simulink model "r2_b16a4x64f"  (R2012b)
settings: Solver=VariableStepDiscrete  SolverMode=SingleTasking  StartTime=0.0  StopTime=1  RelTol=1e-3
undefined symbols (not defined in the file): fft_stages, n_bits_ants, n_bits_xengs
libraries: xbsIndex_r4 x26846, casper_library_misc x230, xbsReplacements_r4 x24, casper_library_delays x8, xps_library x5, casper_library_communications x4
(part 76 of 227)

== system r2_b16a4x64f/sys1/speadify1/spead_pack ==
  note: eof ON the last valid data.
  note: SPEAD header
  note: magic number - 0x53
  note: spead version
  note: item id width in bytes
  note: heap addr width in bytes
  note: <reserved>
  note: num item pointers -
      | after this header
  data64_ready : Inport
  data64_valid : Inport  Port=2
  data64 : Inport  Port=3
  hdr_heap_id : Inport  Port=4
  hdr_heap_size : Inport  Port=5
  hdr_heap_offset : Inport  Port=6
  hdr_pkt_len_words : Inport  Port=7
  hdr5_0x1600_DIR : Inport  Port=8
  hdr6_0x4103_DIR : Inport  Port=9
  hdr7_0x5000 : Inport  Port=10
  AddSub : xbsIndex_r4/AddSub  mode=Subtraction  use_carryin=off  use_carryout=off  en=off  latency=0  precision=Full  arith_type=Unsigned  n_bits=16  bin_pt=14  quantization=Truncate  overflow=Wrap  dbl_ovrd=off  use_behavioral_HDL=off  hw_selection=Fabric  pipelined=off  block_type=addsub
  Assert17 : xbsIndex_r4/Assert  assert_type=on  type_source=Explicitly  gui_display_data_type=Fixed-point  arith_type=Unsigned  n_bits=64  bin_pt=0  preci_type=Single  exp_width=8  frac_width=24  assert_rate=off  rate_source=Explicitly  period=1  output_port=on  block_type=assert
  Assert18 : xbsIndex_r4/Assert  assert_type=on  type_source=Explicitly  gui_display_data_type=Fixed-point  arith_type=Unsigned  n_bits=spead_msw  bin_pt=0  preci_type=Single  exp_width=8  frac_width=24  assert_rate=off  rate_source=Explicitly  period=1  output_port=on  block_type=assert
  Assert5 : xbsIndex_r4/Assert  assert_type=on  type_source=Explicitly  gui_display_data_type=Fixed-point  arith_type=Boolean  n_bits=64  bin_pt=0  preci_type=Single  exp_width=8  frac_width=24  assert_rate=off  rate_source=Explicitly  period=1  output_port=on  block_type=assert
      settings: block_version=10.1.3
  Assert6 : xbsIndex_r4/Assert  assert_type=on  type_source=Explicitly  gui_display_data_type=Fixed-point  arith_type=Unsigned  n_bits=spead_msw  bin_pt=0  preci_type=Single  exp_width=8  frac_width=24  assert_rate=off  rate_source=Explicitly  period=1  output_port=on  block_type=assert
      settings: block_version=10.1.3
  Assert7 : xbsIndex_r4/Assert  assert_type=on  type_source=Explicitly  gui_display_data_type=Boolean  arith_type=Boolean  n_bits=64  bin_pt=0  preci_type=Single  exp_width=8  frac_width=24  assert_rate=off  rate_source=Explicitly  period=1  output_port=on  block_type=assert
      settings: block_version=10.1.3
  Concat : xbsIndex_r4/Concat  num_inputs=6  dbl_ovrd=off  block_type=concat
      settings: block_version=10.1.3
  Constant3 : xbsIndex_r4/Constant  const=83  gui_display_data_type=Fixed-point  arith_type=Unsigned  n_bits=8  bin_pt=0  preci_type=Single  exp_width=8  frac_width=24  explicit_period=on  period=1  equ=P=C  opselect=C  inp2=PCIN>>17  opr=+  inp1=P  carry=CIN  dbl_ovrd=off  block_type=constant
  Constant4 : xbsIndex_r4/Constant  const=spead_version  gui_display_data_type=Fixed-point  arith_type=Unsigned  n_bits=8  bin_pt=0  preci_type=Single  exp_width=8  frac_width=24  explicit_period=on  period=1  equ=P=C  opselect=C  inp2=PCIN>>17  opr=+  inp1=P  carry=CIN  dbl_ovrd=off  block_type=constant
  Constant7 : xbsIndex_r4/Constant  const=0  gui_display_data_type=Fixed-point  arith_type=Unsigned  n_bits=16  bin_pt=0  preci_type=Single  exp_width=8  frac_width=24  explicit_period=on  period=1  equ=P=C  opselect=C  inp2=PCIN>>17  opr=+  inp1=P  carry=CIN  dbl_ovrd=off  block_type=constant
  Delay1 : xbsIndex_r4/Delay  rst=off  infoeditControl=Selection of Reset will increase slice count due to use of real FFs and instead of SRLs  en=off  latency=1  dbl_ovrd=off  reg_retiming=on  block_type=delay
      settings: block_version=11.4
  Delay3 : xbsIndex_r4/Delay  rst=off  infoeditControl=Selection of Reset will increase slice count due to use of real FFs and instead of SRLs  en=off  latency=1  dbl_ovrd=off  reg_retiming=on  block_type=delay
      settings: block_version=11.4
  Logical1 : xbsIndex_r4/Logical  logical_function=AND  inputs=2  en=off  latency=0  precision=Full  arith_type=Unsigned  n_bits=8  bin_pt=2  align_bp=on  dbl_ovrd=off  block_type=logical
      settings: xl_area=[0, 0, 0, 0, 0, 0, 0]
  Logical2 : xbsIndex_r4/Logical  logical_function=AND  inputs=2  en=off  latency=0  precision=Full  arith_type=Unsigned  n_bits=8  bin_pt=2  align_bp=on  dbl_ovrd=off  block_type=logical
      settings: xl_area=[0, 0, 0, 0, 0, 0, 0]
  Logical3 : xbsIndex_r4/Logical  logical_function=OR  inputs=2  en=off  latency=0  precision=Full  arith_type=Unsigned  n_bits=8  bin_pt=2  align_bp=on  dbl_ovrd=off  block_type=logical
      settings: xl_area=[0, 0, 0, 0, 0, 0, 0]
  Logical4 : xbsIndex_r4/Logical  logical_function=AND  inputs=2  en=off  latency=0  precision=Full  arith_type=Unsigned  n_bits=8  bin_pt=2  align_bp=on  dbl_ovrd=off  block_type=logical
      settings: xl_area=[0, 0, 0, 0, 0, 0, 0]
  Register1 : xbsIndex_r4/Register  init=0  rst=on  en=on  dbl_ovrd=off  block_type=register
  Register3 : xbsIndex_r4/Register  init=0  rst=on  en=on  dbl_ovrd=off  block_type=register
  Relational1 : xbsIndex_r4/Relational  mode=a=b  en=off  latency=0  dbl_ovrd=off  block_type=relational
      settings: xl_area=[0, 0, 0, 0, 0, 0, 0]  block_version=10.1.3
  Relational2 : xbsIndex_r4/Relational  mode=a<b  en=off  latency=0  dbl_ovrd=off  block_type=relational
      settings: xl_area=[0, 0, 0, 0, 0, 0, 0]  block_version=10.1.3
  assert_data : xbsIndex_r4/Assert  assert_type=on  type_source=Explicitly  gui_display_data_type=Fixed-point  arith_type=Unsigned  n_bits=spead_msw  bin_pt=0  preci_type=Single  exp_width=8  frac_width=24  assert_rate=off  rate_source=Explicitly  period=1  output_port=on  block_type=assert
  data_ctr : xbsIndex_r4/Counter  cnt_type=Free Running  cnt_to=4  operation=Up  start_count=0  cnt_by_val=1  arith_type=Unsigned  n_bits=max_pkt_len_bits + 1  bin_pt=0  load_pin=off  rst=on  en=on  explicit_period=on  period=1  dbl_ovrd=off  use_behavioral_HDL=off  implementation=Fabric  use_rpm=on  block_type=counter
      settings: xl_area=[0, 0, 0, 0, 0, 0, 0]
  delay_data : xbsIndex_r4/Delay  rst=off  infoeditControl=Selection of Reset will increase slice count due to use of real FFs and instead of SRLs  en=off  latency=8  dbl_ovrd=off  reg_retiming=on  block_type=delay
      settings: block_version=11.4
  delay_data1 : xbsIndex_r4/Delay  rst=off  infoeditControl=Selection of Reset will increase slice count due to use of real FFs and instead of SRLs  en=off  latency=1  dbl_ovrd=off  reg_retiming=on  block_type=delay
      settings: block_version=11.4
  delay_data2 : xbsIndex_r4/Delay  rst=off  infoeditControl=Selection of Reset will increase slice count due to use of real FFs and instead of SRLs  en=off  latency=1  dbl_ovrd=off  reg_retiming=on  block_type=delay
      settings: block_version=11.4
  delay_valid : xbsIndex_r4/Delay  rst=off  infoeditControl=Selection of Reset will increase slice count due to use of real FFs and instead of SRLs  en=off  latency=8  dbl_ovrd=off  reg_retiming=on  block_type=delay
      settings: block_version=11.4
  edge_detect1 : Subsystem  AncestorBlock=casper_library_misc/edge_detect  mask(edge_detect){edge=Rising, polarity=Active High, x_in=[0 0.08 0.08 0.16 0.16 0.24 0.24 0.32 0.32 0.4], y_in=[-1 -1  1  1  1  1  1  1  1  1], x_out=[0.6 0.68 0.68 0.76 0.76 0.84 0.84 0.92 0.92 1], y_out=[-1 -1  1  1 -1 -1 -1 -1 -1 -1]}
      mask prompts: edge "Edge Type"; polarity "Output Polarity"; x_in "Input X Positions"; y_in "Input Y Positions"; x_out "Output X Positions"; y_out "Output Y Positions"
      mask help: Output is active for one-cycle after each edge of the specified type (i.e. rising, falling or both).
      mask init: same as r2_b16a4x64f/edge_detect
      settings: AttributesFormatString=|
      | rising edges
      | active high
      mask Help: Output is active for one-cycle after each edge of the specified type (i.e. rising, falling, or both).  Latency is zero.
      mask TypeOptions edge: Rising | Falling | Both
      mask TypeOptions polarity: Active High | Active Low
      mask Display:
      | plot(x_in_num,0.5+y_in_num*0.2);
      | plot(x_out_num,0.5+y_out_num*0.2);
  edge_detect2 : Subsystem  AncestorBlock=casper_library_misc/edge_detect  mask(edge_detect){edge=Rising, polarity=Active High, x_in=[0 0.08 0.08 0.16 0.16 0.24 0.24 0.32 0.32 0.4], y_in=[-1 -1  1  1  1  1  1  1  1  1], x_out=[0.6 0.68 0.68 0.76 0.76 0.84 0.84 0.92 0.92 1], y_out=[-1 -1  1  1 -1 -1 -1 -1 -1 -1]}
      mask prompts: edge "Edge Type"; polarity "Output Polarity"; x_in "Input X Positions"; y_in "Input Y Positions"; x_out "Output X Positions"; y_out "Output Y Positions"
      mask help: Output is active for one-cycle after each edge of the specified type (i.e. rising, falling or both).
      mask init: same as r2_b16a4x64f/edge_detect
      settings: AttributesFormatString=|
      | rising edges
      | active high
      mask Help: Output is active for one-cycle after each edge of the specified type (i.e. rising, falling, or both).  Latency is zero.
      mask TypeOptions edge: Rising | Falling | Both
      mask TypeOptions polarity: Active High | Active Low
      mask Display:
      | plot(x_in_num,0.5+y_in_num*0.2);
      | plot(x_out_num,0.5+y_out_num*0.2);
  hdr_ctr : xbsIndex_r4/Counter  cnt_type=Count Limited  cnt_to=8  operation=Up  start_count=0  cnt_by_val=1  arith_type=Unsigned  n_bits=4  bin_pt=0  load_pin=off  rst=on  en=on  explicit_period=on  period=1  dbl_ovrd=off  use_behavioral_HDL=off  implementation=Fabric  use_rpm=on  block_type=counter
      settings: xl_area=[0, 0, 0, 0, 0, 0, 0]
  hdra_{1..7} (7 alike) : xbsIndex_r4/Assert  assert_type=on  type_source=Explicitly  gui_display_data_type=Fixed-point  arith_type=Unsigned  n_bits=spead_lsw  bin_pt=0  preci_type=Single  exp_width=8  frac_width=24  assert_rate=off  rate_source=Explicitly  period=1  output_port=on  block_type=assert
  hdrd_1 : xbsIndex_r4/Delay  rst=off  infoeditControl=Selection of Reset will increase slice count due to use of real FFs and instead of SRLs  en=off  latency=2  dbl_ovrd=off  reg_retiming=on  block_type=delay
  hdrd_2 : xbsIndex_r4/Delay  rst=off  infoeditControl=Selection of Reset will increase slice count due to use of real FFs and instead of SRLs  en=off  latency=3  dbl_ovrd=off  reg_retiming=on  block_type=delay
  hdrd_3 : xbsIndex_r4/Delay  rst=off  infoeditControl=Selection of Reset will increase slice count due to use of real FFs and instead of SRLs  en=off  latency=4  dbl_ovrd=off  reg_retiming=on  block_type=delay
  hdrd_4 : xbsIndex_r4/Delay  rst=off  infoeditControl=Selection of Reset will increase slice count due to use of real FFs and instead of SRLs  en=off  latency=5  dbl_ovrd=off  reg_retiming=on  block_type=delay
  hdrd_5 : xbsIndex_r4/Delay  rst=off  infoeditControl=Selection of Reset will increase slice count due to use of real FFs and instead of SRLs  en=off  latency=6  dbl_ovrd=off  reg_retiming=on  block_type=delay
  hdrd_6 : xbsIndex_r4/Delay  rst=off  infoeditControl=Selection of Reset will increase slice count due to use of real FFs and instead of SRLs  en=off  latency=7  dbl_ovrd=off  reg_retiming=on  block_type=delay
  hdrd_7 : xbsIndex_r4/Delay  rst=off  infoeditControl=Selection of Reset will increase slice count due to use of real FFs and instead of SRLs  en=off  latency=8  dbl_ovrd=off  reg_retiming=on  block_type=delay
  header_4cast4 : xbsIndex_r4/Convert  gui_display_data_type=Fixed-point  arith_type=Unsigned  n_bits=spead_lsw - 3  bin_pt=0  float_type=Single  exp_bits=8  fraction_bits=24  quantization=Truncate  overflow=Wrap  en=off  latency=0  dbl_ovrd=off  pipeline=on  block_type=convert
  header_4cat4 : xbsIndex_r4/Concat  num_inputs=2  dbl_ovrd=off  block_type=concat
  header_4const4 : xbsIndex_r4/Constant  const=0  gui_display_data_type=Fixed-point  arith_type=Unsigned  n_bits=3  bin_pt=0  preci_type=Single  exp_width=8  frac_width=24  explicit_period=off  period=1  equ=P=C  opselect=C  inp2=PCIN>>17  opr=+  inp1=P  carry=CIN  dbl_ovrd=off  block_type=constant
  header_assert{1..7} (7 alike) : xbsIndex_r4/Assert  assert_type=on  type_source=Explicitly  gui_display_data_type=Fixed-point  arith_type=Unsigned  n_bits=spead_msw  bin_pt=0  preci_type=Single  exp_width=8  frac_width=24  assert_rate=off  rate_source=Explicitly  period=1  output_port=on  block_type=assert
  header_cat{1..7} (7 alike) : xbsIndex_r4/Concat  num_inputs=2  dbl_ovrd=off  block_type=concat
  header_const1 : xbsIndex_r4/Constant  const=32769  gui_display_data_type=Fixed-point  arith_type=Unsigned  n_bits=spead_msw - spead_lsw  bin_pt=0  preci_type=Single  exp_width=8  frac_width=24  explicit_period=off  period=1  equ=P=C  opselect=C  inp2=PCIN>>17  opr=+  inp1=P  carry=CIN  dbl_ovrd=off  block_type=constant
  header_const2 : xbsIndex_r4/Constant  const=32770  gui_display_data_type=Fixed-point  arith_type=Unsigned  n_bits=spead_msw - spead_lsw  bin_pt=0  preci_type=Single  exp_width=8  frac_width=24  explicit_period=off  period=1  equ=P=C  opselect=C  inp2=PCIN>>17  opr=+  inp1=P  carry=CIN  dbl_ovrd=off  block_type=constant
  header_const3 : xbsIndex_r4/Constant  const=32771  gui_display_data_type=Fixed-point  arith_type=Unsigned  n_bits=spead_msw - spead_lsw  bin_pt=0  preci_type=Single  exp_width=8  frac_width=24  explicit_period=off  period=1  equ=P=C  opselect=C  inp2=PCIN>>17  opr=+  inp1=P  carry=CIN  dbl_ovrd=off  block_type=constant
  header_const4 : xbsIndex_r4/Constant  const=32772  gui_display_data_type=Fixed-point  arith_type=Unsigned  n_bits=spead_msw - spead_lsw  bin_pt=0  preci_type=Single  exp_width=8  frac_width=24  explicit_period=off  period=1  equ=P=C  opselect=C  inp2=PCIN>>17  opr=+  inp1=P  carry=CIN  dbl_ovrd=off  block_type=constant
  header_const5 : xbsIndex_r4/Constant  const=38400  gui_display_data_type=Fixed-point  arith_type=Unsigned  n_bits=spead_msw - spead_lsw  bin_pt=0  preci_type=Single  exp_width=8  frac_width=24  explicit_period=off  period=1  equ=P=C  opselect=C  inp2=PCIN>>17  opr=+  inp1=P  carry=CIN  dbl_ovrd=off  block_type=constant
  header_const6 : xbsIndex_r4/Constant  const=49411  gui_display_data_type=Fixed-point  arith_type=Unsigned  n_bits=spead_msw - spead_lsw  bin_pt=0  preci_type=Single  exp_width=8  frac_width=24  explicit_period=off  period=1  equ=P=C  opselect=C  inp2=PCIN>>17  opr=+  inp1=P  carry=CIN  dbl_ovrd=off  block_type=constant
  header_const7 : xbsIndex_r4/Constant  const=20480  gui_display_data_type=Fixed-point  arith_type=Unsigned  n_bits=spead_msw - spead_lsw  bin_pt=0  preci_type=Single  exp_width=8  frac_width=24  explicit_period=off  period=1  equ=P=C  opselect=C  inp2=PCIN>>17  opr=+  inp1=P  carry=CIN  dbl_ovrd=off  block_type=constant
  heap_addr_width : xbsIndex_r4/Constant  const=spead_lsw/8  gui_display_data_type=Fixed-point  arith_type=Unsigned  n_bits=8  bin_pt=0  preci_type=Single  exp_width=8  frac_width=24  explicit_period=on  period=1  equ=P=C  opselect=C  inp2=PCIN>>17  opr=+  inp1=P  carry=CIN  dbl_ovrd=off  block_type=constant
  item_id_width : xbsIndex_r4/Constant  const=(spead_msw-spead_lsw)/8  gui_display_data_type=Fixed-point  arith_type=Unsigned  n_bits=8  bin_pt=0  preci_type=Single  exp_width=8  frac_width=24  explicit_period=on  period=1  equ=P=C  opselect=C  inp2=PCIN>>17  opr=+  inp1=P  carry=CIN  dbl_ovrd=off  block_type=constant
  mainmux : xbsIndex_r4/Mux  inputs=9  en=off  latency=1  precision=Full  arith_type="Signed  (2's comp)"  n_bits=8  bin_pt=2  quantization=Truncate  overflow=Wrap  dbl_ovrd=off  block_type=mux
      settings: xl_area=[0, 0, 0, 0, 0, 0, 0]
  num_headers : xbsIndex_r4/Constant  const=8  gui_display_data_type=Fixed-point  arith_type=Unsigned  n_bits=4  bin_pt=0  preci_type=Single  exp_width=8  frac_width=24  explicit_period=on  period=1  equ=P=C  opselect=C  inp2=PCIN>>17  opr=+  inp1=P  carry=CIN  dbl_ovrd=off  block_type=constant
  num_item_pts : xbsIndex_r4/Constant  const=7  gui_display_data_type=Fixed-point  arith_type=Unsigned  n_bits=16  bin_pt=0  preci_type=Single  exp_width=8  frac_width=24  explicit_period=on  period=1  equ=P=C  opselect=C  inp2=PCIN>>17  opr=+  inp1=P  carry=CIN  dbl_ovrd=off  block_type=constant
  only_one : xbsIndex_r4/Constant  const=1  gui_display_data_type=Fixed-point  arith_type=Unsigned  n_bits=1  bin_pt=0  preci_type=Single  exp_width=8  frac_width=24  explicit_period=on  period=1  equ=P=C  opselect=C  inp2=PCIN>>17  opr=+  inp1=P  carry=CIN  dbl_ovrd=off  block_type=constant
  data_out : Outport
  valid_out : Outport  Port=2
  eof : Outport  Port=3
  data_overflow : Outport  Port=4
  wires:
  assert_data/1 -> mainmux/10  "pkt_data"
  header_assert7/1 -> mainmux/9
  header_cat7/1 -> header_assert7/1
  [hdr_7] -> header_cat7/2
  header_const7/1 -> header_cat7/1  "spid7"
  hdrd_7/1 -> [hdr_7]
  hdra_7/1 -> hdrd_7/1  "hdr7_0x5000"
  hdr7_0x5000/1 -> hdra_7/1
  header_assert6/1 -> mainmux/8
  header_cat6/1 -> header_assert6/1
  [hdr_6] -> header_cat6/2
  header_const6/1 -> header_cat6/1  "spid6"
  hdrd_6/1 -> [hdr_6]
  hdra_6/1 -> hdrd_6/1  "hdr6_0x4103_DIR"
  hdr6_0x4103_DIR/1 -> hdra_6/1
  header_assert5/1 -> mainmux/7
  header_cat5/1 -> header_assert5/1
  [hdr_5] -> header_cat5/2
  header_const5/1 -> header_cat5/1  "spid5"
  hdrd_5/1 -> [hdr_5]
  hdra_5/1 -> hdrd_5/1  "hdr5_0x1600_DIR"
  hdr5_0x1600_DIR/1 -> hdra_5/1
  header_assert4/1 -> mainmux/6
  header_cat4/1 -> header_assert4/1
  header_4cat4/1 -> header_cat4/2
  header_4const4/1 -> header_4cat4/2
  header_4cast4/1 -> header_4cat4/1
  [hdr_4] -> header_4cast4/1
  header_const4/1 -> header_cat4/1  "spid4"
  hdrd_4/1 -> [hdr_4]
  hdra_4/1 -> hdrd_4/1  "hdr_pkt_len_words"
  hdr_pkt_len_words/1 -> hdra_4/1
  header_assert3/1 -> mainmux/5
  header_cat3/1 -> header_assert3/1
  [hdr_3] -> header_cat3/2
  header_const3/1 -> header_cat3/1  "spid3"
  hdrd_3/1 -> [hdr_3]
  hdra_3/1 -> hdrd_3/1  "hdr_heap_offset"
  hdr_heap_offset/1 -> hdra_3/1
  header_assert2/1 -> mainmux/4
  header_cat2/1 -> header_assert2/1
  [hdr_2] -> header_cat2/2
  header_const2/1 -> header_cat2/1  "spid2"
  hdrd_2/1 -> [hdr_2]
  hdra_2/1 -> hdrd_2/1  "hdr_heap_size"
  hdr_heap_size/1 -> hdra_2/1
  header_assert1/1 -> mainmux/3
  header_cat1/1 -> header_assert1/1
  [hdr_1] -> header_cat1/2
  header_const1/1 -> header_cat1/1  "spid1"
  hdrd_1/1 -> [hdr_1]
  hdra_1/1 -> hdrd_1/1  "hdr_heap_id"
  hdr_heap_id/1 -> hdra_1/1
  Logical4/1 -> data_overflow/1  "overflow"
  [new_sync] -> Logical4/2
  delay_data2/1 -> delay_valid/1
  delay_data1/1 -> delay_data/1
  Logical2/1 -> [new_sync]  "new_sync"
  edge_detect2/1(out) -> Register1/2, Logical2/2
  Register1/1 -> Logical2/1  "armed"
  Delay3/1 -> eof/1  "eof_out"
  Relational1/1 -> Delay3/1  "eof_real"
  AddSub/1 -> Relational1/2
  data_ctr/1 -> Relational1/1  "data_ctr"
  [new_sync] -> data_ctr/1
  [writing_pld] -> data_ctr/2
  edge_detect1/1(out) -> Register3/2  "rst"
  num_item_pts/1 -> Concat/6
  Assert18/1 -> data_out/1
  Assert17/1 -> mainmux/2
  [pkt_data] -> assert_data/1
  Logical1/1 -> [writing_header]  "w_hdr"
  Relational2/1 -> Logical1/1  "wr_header"
  Register3/1 -> Logical1/2  "armed"
  [new_sync] -> Register3/1, Register3/3
  Delay1/1 -> valid_out/1  "valid"
  Assert7/1 -> delay_data2/1, edge_detect2/1(in)  "data64_valid"
  data64_valid/1 -> Assert7/1
  [writing_pld] -> Logical3/2
  [writing_header] -> Logical3/1
  Logical3/1 -> Delay1/1, Logical4/1  "busy"
  [new_sync] -> hdr_ctr/1
  [writing_header] -> hdr_ctr/2
  num_headers/1 -> Relational2/2
  data64_ready/1 -> Assert5/1
  Assert5/1 -> Register1/1, Register1/3  "data64_rdy"
  Assert6/1 -> delay_data1/1  "data64"
  data64/1 -> Assert6/1
  [output_select] -> mainmux/1
  hdr_ctr/1 -> [output_select], Relational2/1  "output_sel"
  mainmux/1 -> Assert18/1  "dout"
  Constant7/1 -> Concat/5
  heap_addr_width/1 -> Concat/4
  item_id_width/1 -> Concat/3
  Constant4/1 -> Concat/2
  Constant3/1 -> Concat/1
  Concat/1 -> Assert17/1  "spd_hdr"
  delay_data/1 -> [pkt_data]  "d64"
  delay_valid/1 -> [writing_pld], edge_detect1/1(in)  "wr_pld"
  only_one/1 -> AddSub/2
  [hdr_4] -> AddSub/1

== system r2_b16a4x64f/sys1/tagger_and_flagger/bus_replicate ==
  in : Inport
  bussify : Subsystem  AncestorBlock=casper_library_flow_control/bus_create  mask(bus_create){inputNum=19}
      mask prompts: inputNum "Number of inputs:"
      mask init:
      | bus_create_init(gcb,...
      |     'inputNum', inputNum);
  out : Outport
  wires:
  bussify/1(bus_out) -> out/1
  in/1 -> bussify/19(in19), bussify/18(in18), bussify/17(in17), bussify/16(in16), bussify/15(in15), bussify/14(in14), bussify/13(in13), bussify/12(in12), bussify/11(in11), bussify/10(in10), bussify/9(in9), bussify/8(in8), bussify/7(in7), bussify/6(in6), bussify/5(in5), bussify/4(in4), bussify/3(in3), bussify/2(in2), bussify/1(in1)

== system r2_b16a4x64f/sys1/tagger_and_flagger/flag_register ==
  din : Inport
  rst : Inport  Port=2
  en : Inport  Port=3
  din_expand : Subsystem  AncestorBlock=casper_library_flow_control/bus_expand  mask(bus_expand){mode=divisions of arbitrary size, outputNum=1, outputWidth=[1  1  1  1  1  1  1  1  1  1  1  1  1  1  1  1  1  1  1], outputBinaryPt=[0  0  0  0  0  0  0  0  0  0  0  0  0  0  0  0  0  0  0], outputArithmeticType=[0  0  0  0  0  0  0  0  0  0  0  0  0  0  0  0  0  0  0], show_format=on, outputToWorkspace=off, variablePrefix=, outputToModelAsWell=on}
      mask prompts: outputNum "Number of outputs:"; outputWidth "Output width [msb ... lsb]:"; outputBinaryPt "Output binary point position [msb ... lsb]:"; outputArithmeticType "Output arithmetic type (ufix=0, fix=1, bool=2) [msb ... lsb]:"; show_format "Print format string?"; outputToWorkspace "Output to workspace?"; variablePrefix "Variable name prefix:"; outputToModelAsWell "Output to model as well?"
      mask help:
      | Expands a 'bus' made using a bus_create or Xilinx
      | concat block.
      | The input will be divided into the specified number
      | of outputs with the specified arithmetic types.
      | Divisions are made from most significant bit.
      mask init: same as r2_b16a4x64f/bus_expand
      settings: AttributesFormatString=19 outputs: uf1.0,uf1.0,uf1.0,uf1.0,uf1.0,uf1.0,uf1.0,uf1.0,uf1.0,uf1.0,uf1.0,uf1.0,uf1.0,uf1.0,uf1.0,uf1.0,uf1.0,uf1.0,uf1.0,
      mask TypeOptions mode: divisions of equal size | divisions of arbitrary size
      mask Callback mode: bus_expand_callback();
      mask Callback outputWidth: bus_expand_callback();
      mask Callback outputToWorkspace: bus_expand_callback();
  dout_compress : Subsystem  AncestorBlock=casper_library_flow_control/bus_create  mask(bus_create){inputNum=19}
      mask prompts: inputNum "Number of inputs:"
      mask init:
      | bus_create_init(gcb,...
      |     'inputNum', inputNum);
  en_expand : Subsystem  AncestorBlock=casper_library_flow_control/bus_expand  mask(bus_expand){mode=divisions of equal size, outputNum=19, outputWidth=1, outputBinaryPt=0, outputArithmeticType=2, show_format=on, outputToWorkspace=off, variablePrefix=, outputToModelAsWell=on}
      mask prompts: outputNum "Number of outputs:"; outputWidth "Output width:"; outputBinaryPt "Output binary point position:"; outputArithmeticType "Output arithmetic type (ufix=0, fix=1, bool=2):"; show_format "Print format string?"; outputToWorkspace "Output to workspace?"; variablePrefix "Variable name prefix:"; outputToModelAsWell "Output to model as well?"
      mask help:
      | Expands a 'bus' made using a bus_create or Xilinx
      | concat block.
      | The input will be divided into the specified number
      | of outputs with the specified arithmetic types.
      | Divisions are made from most significant bit.
      mask init: same as r2_b16a4x64f/bus_expand
      settings: AttributesFormatString=19 outputs: b,b,b,b,b,b,b,b,b,b,b,b,b,b,b,b,b,b,b,
      mask TypeOptions mode: divisions of equal size | divisions of arbitrary size
      mask Callback mode: bus_expand_callback();
      mask Callback outputWidth: bus_expand_callback();
      mask Callback outputToWorkspace: bus_expand_callback();
  reg{1..19} (19 alike) : xbsIndex_r4/Register  init=0  rst=on  en=on  dbl_ovrd=off  block_type=register
  rst_expand : Subsystem  AncestorBlock=casper_library_flow_control/bus_expand  mask(bus_expand){mode=divisions of equal size, outputNum=19, outputWidth=1, outputBinaryPt=0, outputArithmeticType=2, show_format=on, outputToWorkspace=off, variablePrefix=, outputToModelAsWell=on}
      mask prompts: outputNum "Number of outputs:"; outputWidth "Output width:"; outputBinaryPt "Output binary point position:"; outputArithmeticType "Output arithmetic type (ufix=0, fix=1, bool=2):"; show_format "Print format string?"; outputToWorkspace "Output to workspace?"; variablePrefix "Variable name prefix:"; outputToModelAsWell "Output to model as well?"
      mask help:
      | Expands a 'bus' made using a bus_create or Xilinx
      | concat block.
      | The input will be divided into the specified number
      | of outputs with the specified arithmetic types.
      | Divisions are made from most significant bit.
      mask init: same as r2_b16a4x64f/bus_expand
      settings: AttributesFormatString=19 outputs: b,b,b,b,b,b,b,b,b,b,b,b,b,b,b,b,b,b,b,
      mask TypeOptions mode: divisions of equal size | divisions of arbitrary size
      mask Callback mode: bus_expand_callback();
      mask Callback outputWidth: bus_expand_callback();
      mask Callback outputToWorkspace: bus_expand_callback();
  dout : Outport
  wires:
  dout_compress/1(bus_out) -> dout/1
  reg19/1 -> dout_compress/19(in19)
  reg18/1 -> dout_compress/18(in18)
  reg17/1 -> dout_compress/17(in17)
  reg16/1 -> dout_compress/16(in16)
  reg15/1 -> dout_compress/15(in15)
  reg14/1 -> dout_compress/14(in14)
  reg13/1 -> dout_compress/13(in13)
  reg12/1 -> dout_compress/12(in12)
  reg11/1 -> dout_compress/11(in11)
  reg10/1 -> dout_compress/10(in10)
  reg9/1 -> dout_compress/9(in9)
  reg8/1 -> dout_compress/8(in8)
  reg7/1 -> dout_compress/7(in7)
  reg6/1 -> dout_compress/6(in6)
  reg5/1 -> dout_compress/5(in5)
  reg4/1 -> dout_compress/4(in4)
  reg3/1 -> dout_compress/3(in3)
  reg2/1 -> dout_compress/2(in2)
  reg1/1 -> dout_compress/1(in1)
  en_expand/19(lsb_out1) -> reg19/3
  rst_expand/19(lsb_out1) -> reg19/2
  din_expand/19(lsb_out1) -> reg19/1
  en_expand/18(out2) -> reg18/3
  rst_expand/18(out2) -> reg18/2
  din_expand/18(out2) -> reg18/1
  en_expand/17(out3) -> reg17/3
  rst_expand/17(out3) -> reg17/2
  din_expand/17(out3) -> reg17/1
  en_expand/16(out4) -> reg16/3
  rst_expand/16(out4) -> reg16/2
  din_expand/16(out4) -> reg16/1
  en_expand/15(out5) -> reg15/3
  rst_expand/15(out5) -> reg15/2
  din_expand/15(out5) -> reg15/1
  en_expand/14(out6) -> reg14/3
  rst_expand/14(out6) -> reg14/2
  din_expand/14(out6) -> reg14/1
  en_expand/13(out7) -> reg13/3
  rst_expand/13(out7) -> reg13/2
  din_expand/13(out7) -> reg13/1
  en_expand/12(out8) -> reg12/3
  rst_expand/12(out8) -> reg12/2
  din_expand/12(out8) -> reg12/1
  en_expand/11(out9) -> reg11/3
  rst_expand/11(out9) -> reg11/2
  din_expand/11(out9) -> reg11/1
  en_expand/10(out10) -> reg10/3
  rst_expand/10(out10) -> reg10/2
  din_expand/10(out10) -> reg10/1
  en_expand/9(out11) -> reg9/3
  rst_expand/9(out11) -> reg9/2
  din_expand/9(out11) -> reg9/1
  en_expand/8(out12) -> reg8/3
  rst_expand/8(out12) -> reg8/2
  din_expand/8(out12) -> reg8/1
  en_expand/7(out13) -> reg7/3
  rst_expand/7(out13) -> reg7/2
  din_expand/7(out13) -> reg7/1
  en_expand/6(out14) -> reg6/3
  rst_expand/6(out14) -> reg6/2
  din_expand/6(out14) -> reg6/1
  en_expand/5(out15) -> reg5/3
  rst_expand/5(out15) -> reg5/2
  din_expand/5(out15) -> reg5/1
  en_expand/4(out16) -> reg4/3
  rst_expand/4(out16) -> reg4/2
  din_expand/4(out16) -> reg4/1
  en_expand/3(out17) -> reg3/3
  rst_expand/3(out17) -> reg3/2
  din_expand/3(out17) -> reg3/1
  en_expand/2(out18) -> reg2/3
  rst_expand/2(out18) -> reg2/2
  din_expand/2(out18) -> reg2/1
  en_expand/1(msb_out19) -> reg1/3
  rst_expand/1(msb_out19) -> reg1/2
  din_expand/1(msb_out19) -> reg1/1
  en/1 -> en_expand/1(bus_in)
  rst/1 -> rst_expand/1(bus_in)
  din/1 -> din_expand/1(bus_in)

== system r2_b16a4x64f/sys1/tl_reord_flags/control ==
  sim_1 : Inport
  io_delay : xbsIndex_r4/Delay  rst=off  infoeditControl=Selection of Reset will increase slice count due to use of real FFs and instead of SRLs  en=off  latency=0  dbl_ovrd=off  reg_retiming=on  block_type=delay
  r2_b16a4x64f_sys1_tl_reord_flags_control_user_data_out : xbsIndex_r4/Gateway In  gui_display_data_type=Fixed-point  arith_type=Unsigned  n_bits=32  bin_pt=0  preci_type=Single  exp_width=8  frac_width=24  quantization="Round  (unbiased: +/- Inf)"  overflow=Saturate  period=1  dbl_ovrd=off  timing_constraint=None  locs_specified=off  LOCs={}  UseAsADC=off  ADCChannel='1'  inherit_from_input=off  hdl_port=on  block_type=gatewayin
  reint1 : xbsIndex_r4/Reinterpret  force_arith_type=on  arith_type=Unsigned  force_bin_pt=on  bin_pt=0  block_type=reinterpret
  slice_load_time_lsw : xbsIndex_r4/Slice  nbits=32  boolean_output=off  mode=Lower Bit Location + Width  bit1=0  base1=MSB of Input  bit0=0  base0=LSB of Input  dbl_ovrd=off  block_type=slice
  in_load_time_lsw : Outport
  wires:
  r2_b16a4x64f_sys1_tl_reord_flags_control_user_data_out/1 -> io_delay/1
  sim_1/1 -> r2_b16a4x64f_sys1_tl_reord_flags_control_user_data_out/1
  io_delay/1 -> slice_load_time_lsw/1
  slice_load_time_lsw/1 -> reint1/1
  reint1/1 -> in_load_time_lsw/1

== system r2_b16a4x64f/sys1/tl_reord_flags/control0 ==
  convert1_1 : DataTypeConversion  OutDataTypeStr=fixdt('ufix1_En0')  LockScale=on
  convert1_2 : DataTypeConversion  OutDataTypeStr=fixdt('ufix1_En0')  LockScale=on
  convert1_3 : DataTypeConversion  OutDataTypeStr=fixdt('ufix16_En0')  LockScale=on
  convert2_1 : DataTypeConversion  OutDataTypeStr=fixdt('ufix1_En0')  ConvertRealWorld=Stored Integer (SI)  LockScale=on
  convert2_2 : DataTypeConversion  OutDataTypeStr=fixdt('ufix1_En0')  ConvertRealWorld=Stored Integer (SI)  LockScale=on
  convert2_3 : DataTypeConversion  OutDataTypeStr=fixdt('ufix16_En0')  ConvertRealWorld=Stored Integer (SI)  LockScale=on
  gain_1 : Gain  Gain=131072
  gain_2 : Gain  Gain=65536
  gain_3 : Gain
  io_delay : xbsIndex_r4/Delay  rst=off  infoeditControl=Selection of Reset will increase slice count due to use of real FFs and instead of SRLs  en=off  latency=0  dbl_ovrd=off  reg_retiming=on  block_type=delay
  r2_b16a4x64f_sys1_tl_reord_flags_control0_user_data_out : xbsIndex_r4/Gateway In  gui_display_data_type=Fixed-point  arith_type=Unsigned  n_bits=32  bin_pt=0  preci_type=Single  exp_width=8  frac_width=24  quantization="Round  (unbiased: +/- Inf)"  overflow=Saturate  period=1  dbl_ovrd=off  timing_constraint=None  locs_specified=off  LOCs={}  UseAsADC=off  ADCChannel='1'  inherit_from_input=off  hdl_port=on  block_type=gatewayin
  reint3 : xbsIndex_r4/Reinterpret  force_arith_type=on  arith_type=Unsigned  force_bin_pt=on  bin_pt=0  block_type=reinterpret
  sim_1 : Constant  Value=0
  sim_2 : Constant  Value=0
  sim_3 : Constant  Value=0
  sim_add : Sum  Inputs=+++  OutDataTypeStr=uint32
  slice_arm : xbsIndex_r4/Slice  nbits=1  boolean_output=on  mode=Lower Bit Location + Width  bit1=0  base1=MSB of Input  bit0=17  base0=LSB of Input  dbl_ovrd=off  block_type=slice
  slice_load_immediate : xbsIndex_r4/Slice  nbits=1  boolean_output=on  mode=Lower Bit Location + Width  bit1=0  base1=MSB of Input  bit0=16  base0=LSB of Input  dbl_ovrd=off  block_type=slice
  slice_load_time_msw : xbsIndex_r4/Slice  nbits=16  boolean_output=off  mode=Lower Bit Location + Width  bit1=0  base1=MSB of Input  bit0=0  base0=LSB of Input  dbl_ovrd=off  block_type=slice
  in_arm : Outport
  in_load_immediate : Outport  Port=2
  in_load_time_msw : Outport  Port=3
  wires:
  r2_b16a4x64f_sys1_tl_reord_flags_control0_user_data_out/1 -> io_delay/1
  sim_add/1 -> r2_b16a4x64f_sys1_tl_reord_flags_control0_user_data_out/1
  sim_1/1 -> convert1_1/1
  convert1_1/1 -> convert2_1/1
  convert2_1/1 -> gain_1/1
  gain_1/1 -> sim_add/1
  io_delay/1 -> slice_arm/1, slice_load_immediate/1, slice_load_time_msw/1
  slice_arm/1 -> in_arm/1
  sim_2/1 -> convert1_2/1
  convert1_2/1 -> convert2_2/1
  convert2_2/1 -> gain_2/1
  gain_2/1 -> sim_add/2
  slice_load_immediate/1 -> in_load_immediate/1
  sim_3/1 -> convert1_3/1
  convert1_3/1 -> convert2_3/1
  convert2_3/1 -> gain_3/1
  gain_3/1 -> sim_add/3
  slice_load_time_msw/1 -> reint3/1
  reint3/1 -> in_load_time_msw/1

== system r2_b16a4x64f/sys1/tl_reord_flags/edge_detect ==
  in : Inport
  Delay : xbsIndex_r4/Delay  rst=off  infoeditControl=Selection of Reset will increase slice count due to use of real FFs and instead of SRLs  en=off  latency=1  dbl_ovrd=off  reg_retiming=on  block_type=delay
      settings: xl_area=[0, 0, 0, 0, 0, 0, 0]
  Inverter : xbsIndex_r4/Inverter  en=off  latency=0  dbl_ovrd=off  block_type=inv
      settings: xl_area=[0, 0, 0, 0, 0, 0, 0]
  edge_op : xbsIndex_r4/Logical  logical_function=NOR  inputs=2  en=off  latency=0  precision=Full  arith_type=Unsigned  n_bits=8  bin_pt=2  align_bp=on  dbl_ovrd=off  block_type=logical
      settings: xl_area=[0, 0, 0, 0, 0, 0, 0]
  out : Outport
  wires:
  Delay/1 -> edge_op/2
  in/1 -> Delay/1, Inverter/1
  edge_op/1 -> out/1
  Inverter/1 -> edge_op/1

== system r2_b16a4x64f/sys1/tl_reord_flags/edge_detect1 ==
  in : Inport
  Delay : xbsIndex_r4/Delay  rst=off  infoeditControl=Selection of Reset will increase slice count due to use of real FFs and instead of SRLs  en=off  latency=1  dbl_ovrd=off  reg_retiming=on  block_type=delay
      settings: xl_area=[0, 0, 0, 0, 0, 0, 0]
  Inverter : xbsIndex_r4/Inverter  en=off  latency=0  dbl_ovrd=off  block_type=inv
      settings: xl_area=[0, 0, 0, 0, 0, 0, 0]
  edge_op : xbsIndex_r4/Logical  logical_function=NOR  inputs=2  en=off  latency=0  precision=Full  arith_type=Unsigned  n_bits=8  bin_pt=2  align_bp=on  dbl_ovrd=off  block_type=logical
      settings: xl_area=[0, 0, 0, 0, 0, 0, 0]
  out : Outport
  wires:
  Delay/1 -> edge_op/2
  in/1 -> Delay/1, Inverter/1
  edge_op/1 -> out/1
  Inverter/1 -> edge_op/1

== system r2_b16a4x64f/sys1/tl_reord_flags/pipeline ==
  d : Inport
  Register0 : xbsIndex_r4/Register  init=0  rst=off  en=off  dbl_ovrd=off  block_type=register
      settings: block_version=11.4
  Register1 : xbsIndex_r4/Register  init=0  rst=off  en=off  dbl_ovrd=off  block_type=register
      settings: block_version=11.4
  q : Outport
  wires:
  Register1/1 -> q/1
  d/1 -> Register0/1
  Register0/1 -> Register1/1

== system r2_b16a4x64f/sys1/tl_reord_flags/pipeline1 ==
  d : Inport
  Register0 : xbsIndex_r4/Register  init=0  rst=off  en=off  dbl_ovrd=off  block_type=register
      settings: block_version=11.4
  Register1 : xbsIndex_r4/Register  init=0  rst=off  en=off  dbl_ovrd=off  block_type=register
      settings: block_version=11.4
  q : Outport
  wires:
  Register0/1 -> Register1/1
  d/1 -> Register0/1
  Register1/1 -> q/1

== system r2_b16a4x64f/sys1/tl_reord_flags/pipeline2 ==
  d : Inport
  Register0 : xbsIndex_r4/Register  init=0  rst=off  en=off  dbl_ovrd=off  block_type=register
      settings: block_version=11.4
  Register1 : xbsIndex_r4/Register  init=0  rst=off  en=off  dbl_ovrd=off  block_type=register
      settings: block_version=11.4
  q : Outport
  wires:
  Register1/1 -> q/1
  d/1 -> Register0/1
  Register0/1 -> Register1/1

== system r2_b16a4x64f/sys1/tl_reord_flags/pipeline3 ==
  d : Inport
  Register0 : xbsIndex_r4/Register  init=0  rst=off  en=off  dbl_ovrd=off  block_type=register
      settings: block_version=11.4
  Register1 : xbsIndex_r4/Register  init=0  rst=off  en=off  dbl_ovrd=off  block_type=register
      settings: block_version=11.4
  q : Outport
  wires:
  Register0/1 -> Register1/1
  d/1 -> Register0/1
  Register1/1 -> q/1

== system r2_b16a4x64f/sys1/tl_reord_flags/pipeline4 ==
  d : Inport
  Register0 : xbsIndex_r4/Register  init=0  rst=off  en=off  dbl_ovrd=off  block_type=register
      settings: block_version=11.4
  Register1 : xbsIndex_r4/Register  init=0  rst=off  en=off  dbl_ovrd=off  block_type=register
      settings: block_version=11.4
  q : Outport
  wires:
  Register1/1 -> q/1
  d/1 -> Register0/1
  Register0/1 -> Register1/1

== system r2_b16a4x64f/sys1/tl_reord_flags/pipeline5 ==
  d : Inport
  Register0 : xbsIndex_r4/Register  init=0  rst=off  en=off  dbl_ovrd=off  block_type=register
      settings: block_version=11.4
  Register1 : xbsIndex_r4/Register  init=0  rst=off  en=off  dbl_ovrd=off  block_type=register
      settings: block_version=11.4
  q : Outport
  wires:
  Register1/1 -> q/1
  d/1 -> Register0/1
  Register0/1 -> Register1/1

== system r2_b16a4x64f/sys1/tl_reord_flags/status ==
  out_armed : Inport
  out_arm_count : Inport  Port=2
  out_load_count : Inport  Port=3
  assert_arm_count : xbsIndex_r4/Assert  assert_type=on  type_source=Explicitly  gui_display_data_type=Fixed-point  arith_type=Unsigned  n_bits=8  bin_pt=0  preci_type=Single  exp_width=8  frac_width=24  assert_rate=off  rate_source=Explicitly  period=1  output_port=on  block_type=assert
  assert_armed : xbsIndex_r4/Assert  assert_type=on  type_source=Explicitly  gui_display_data_type=Boolean  arith_type=Boolean  n_bits=1  bin_pt=0  preci_type=Single  exp_width=8  frac_width=24  assert_rate=off  rate_source=Explicitly  period=1  output_port=on  block_type=assert
  assert_load_count : xbsIndex_r4/Assert  assert_type=on  type_source=Explicitly  gui_display_data_type=Fixed-point  arith_type=Unsigned  n_bits=8  bin_pt=0  preci_type=Single  exp_width=8  frac_width=24  assert_rate=off  rate_source=Explicitly  period=1  output_port=on  block_type=assert
  cast_gw : xbsIndex_r4/Convert  gui_display_data_type=Fixed-point  arith_type=Unsigned  n_bits=32  bin_pt=0  float_type=Single  exp_bits=8  fraction_bits=24  quantization=Truncate  overflow=Wrap  en=off  latency=0  dbl_ovrd=off  pipeline=off  block_type=convert
  concatenate : xbsIndex_r4/Concat  num_inputs=3  dbl_ovrd=off  block_type=concat
  io_delay : xbsIndex_r4/Delay  rst=off  infoeditControl=Selection of Reset will increase slice count due to use of real FFs and instead of SRLs  en=off  latency=1  dbl_ovrd=off  reg_retiming=on  block_type=delay
  r2_b16a4x64f_sys1_tl_reord_flags_status_user_data_in : xbsIndex_r4/Gateway Out  inherit_from_input=off  hdl_port=on  timing_constraint=None  locs_specified=off  LOCs={}  UseAsDAC=off  DACChannel='1'  block_type=gatewayout
  reint1 : xbsIndex_r4/Reinterpret  force_arith_type=on  arith_type=Unsigned  force_bin_pt=on  bin_pt=0  block_type=reinterpret
  reint2 : xbsIndex_r4/Reinterpret  force_arith_type=on  arith_type=Unsigned  force_bin_pt=on  bin_pt=0  block_type=reinterpret
  reint3 : xbsIndex_r4/Reinterpret  force_arith_type=on  arith_type=Unsigned  force_bin_pt=on  bin_pt=0  block_type=reinterpret
  sim_out : Terminator
  wires:
  concatenate/1 -> io_delay/1
  io_delay/1 -> cast_gw/1
  cast_gw/1 -> r2_b16a4x64f_sys1_tl_reord_flags_status_user_data_in/1
  r2_b16a4x64f_sys1_tl_reord_flags_status_user_data_in/1 -> sim_out/1
  out_armed/1 -> assert_armed/1
  assert_armed/1 -> reint1/1
  reint1/1 -> concatenate/1
  out_arm_count/1 -> assert_arm_count/1
  assert_arm_count/1 -> reint2/1
  reint2/1 -> concatenate/2
  out_load_count/1 -> assert_load_count/1
  assert_load_count/1 -> reint3/1
  reint3/1 -> concatenate/3

== system r2_b16a4x64f/sys1/vacc/bus_register ==
  din : Inport
  rst : Inport  Port=2
  en : Inport  Port=3
  din_expand : Subsystem  AncestorBlock=casper_library_flow_control/bus_expand  mask(bus_expand){mode=divisions of arbitrary size, outputNum=1, outputWidth=[1  1  1  1  1  1  1  1  1  1  1  1  1  1  1  1  1  1  1], outputBinaryPt=[0  0  0  0  0  0  0  0  0  0  0  0  0  0  0  0  0  0  0], outputArithmeticType=[0  0  0  0  0  0  0  0  0  0  0  0  0  0  0  0  0  0  0], show_format=on, outputToWorkspace=off, variablePrefix=, outputToModelAsWell=on}
      mask prompts: outputNum "Number of outputs:"; outputWidth "Output width [msb ... lsb]:"; outputBinaryPt "Output binary point position [msb ... lsb]:"; outputArithmeticType "Output arithmetic type (ufix=0, fix=1, bool=2) [msb ... lsb]:"; show_format "Print format string?"; outputToWorkspace "Output to workspace?"; variablePrefix "Variable name prefix:"; outputToModelAsWell "Output to model as well?"
      mask help:
      | Expands a 'bus' made using a bus_create or Xilinx
      | concat block.
      | The input will be divided into the specified number
      | of outputs with the specified arithmetic types.
      | Divisions are made from most significant bit.
      mask init: same as r2_b16a4x64f/bus_expand
      settings: AttributesFormatString=19 outputs: uf1.0,uf1.0,uf1.0,uf1.0,uf1.0,uf1.0,uf1.0,uf1.0,uf1.0,uf1.0,uf1.0,uf1.0,uf1.0,uf1.0,uf1.0,uf1.0,uf1.0,uf1.0,uf1.0,
      mask TypeOptions mode: divisions of equal size | divisions of arbitrary size
      mask Callback mode: bus_expand_callback();
      mask Callback outputWidth: bus_expand_callback();
      mask Callback outputToWorkspace: bus_expand_callback();
  dout_compress : Subsystem  AncestorBlock=casper_library_flow_control/bus_create  mask(bus_create){inputNum=19}
      mask prompts: inputNum "Number of inputs:"
      mask init:
      | bus_create_init(gcb,...
      |     'inputNum', inputNum);
  en_expand : Subsystem  AncestorBlock=casper_library_flow_control/bus_expand  mask(bus_expand){mode=divisions of equal size, outputNum=19, outputWidth=1, outputBinaryPt=0, outputArithmeticType=2, show_format=on, outputToWorkspace=off, variablePrefix=, outputToModelAsWell=on}
      mask prompts: outputNum "Number of outputs:"; outputWidth "Output width:"; outputBinaryPt "Output binary point position:"; outputArithmeticType "Output arithmetic type (ufix=0, fix=1, bool=2):"; show_format "Print format string?"; outputToWorkspace "Output to workspace?"; variablePrefix "Variable name prefix:"; outputToModelAsWell "Output to model as well?"
      mask help:
      | Expands a 'bus' made using a bus_create or Xilinx
      | concat block.
      | The input will be divided into the specified number
      | of outputs with the specified arithmetic types.
      | Divisions are made from most significant bit.
      mask init: same as r2_b16a4x64f/bus_expand
      settings: AttributesFormatString=19 outputs: b,b,b,b,b,b,b,b,b,b,b,b,b,b,b,b,b,b,b,
      mask TypeOptions mode: divisions of equal size | divisions of arbitrary size
      mask Callback mode: bus_expand_callback();
      mask Callback outputWidth: bus_expand_callback();
      mask Callback outputToWorkspace: bus_expand_callback();
  reg{1..19} (19 alike) : xbsIndex_r4/Register  init=0  rst=on  en=on  dbl_ovrd=off  block_type=register
  rst_expand : Subsystem  AncestorBlock=casper_library_flow_control/bus_expand  mask(bus_expand){mode=divisions of equal size, outputNum=19, outputWidth=1, outputBinaryPt=0, outputArithmeticType=2, show_format=on, outputToWorkspace=off, variablePrefix=, outputToModelAsWell=on}
      mask prompts: outputNum "Number of outputs:"; outputWidth "Output width:"; outputBinaryPt "Output binary point position:"; outputArithmeticType "Output arithmetic type (ufix=0, fix=1, bool=2):"; show_format "Print format string?"; outputToWorkspace "Output to workspace?"; variablePrefix "Variable name prefix:"; outputToModelAsWell "Output to model as well?"
      mask help:
      | Expands a 'bus' made using a bus_create or Xilinx
      | concat block.
      | The input will be divided into the specified number
      | of outputs with the specified arithmetic types.
      | Divisions are made from most significant bit.
      mask init: same as r2_b16a4x64f/bus_expand
      settings: AttributesFormatString=19 outputs: b,b,b,b,b,b,b,b,b,b,b,b,b,b,b,b,b,b,b,
      mask TypeOptions mode: divisions of equal size | divisions of arbitrary size
      mask Callback mode: bus_expand_callback();
      mask Callback outputWidth: bus_expand_callback();
      mask Callback outputToWorkspace: bus_expand_callback();
  dout : Outport
  wires:
  dout_compress/1(bus_out) -> dout/1
  reg19/1 -> dout_compress/19(in19)
  reg18/1 -> dout_compress/18(in18)
  reg17/1 -> dout_compress/17(in17)
  reg16/1 -> dout_compress/16(in16)
  reg15/1 -> dout_compress/15(in15)
  reg14/1 -> dout_compress/14(in14)
  reg13/1 -> dout_compress/13(in13)
  reg12/1 -> dout_compress/12(in12)
  reg11/1 -> dout_compress/11(in11)
  reg10/1 -> dout_compress/10(in10)
  reg9/1 -> dout_compress/9(in9)
  reg8/1 -> dout_compress/8(in8)
  reg7/1 -> dout_compress/7(in7)
  reg6/1 -> dout_compress/6(in6)
  reg5/1 -> dout_compress/5(in5)
  reg4/1 -> dout_compress/4(in4)
  reg3/1 -> dout_compress/3(in3)
  reg2/1 -> dout_compress/2(in2)
  reg1/1 -> dout_compress/1(in1)
  en_expand/19(lsb_out1) -> reg19/3
  rst_expand/19(lsb_out1) -> reg19/2
  din_expand/19(lsb_out1) -> reg19/1
  en_expand/18(out2) -> reg18/3
  rst_expand/18(out2) -> reg18/2
  din_expand/18(out2) -> reg18/1
  en_expand/17(out3) -> reg17/3
  rst_expand/17(out3) -> reg17/2
  din_expand/17(out3) -> reg17/1
  en_expand/16(out4) -> reg16/3
  rst_expand/16(out4) -> reg16/2
  din_expand/16(out4) -> reg16/1
  en_expand/15(out5) -> reg15/3
  rst_expand/15(out5) -> reg15/2
  din_expand/15(out5) -> reg15/1
  en_expand/14(out6) -> reg14/3
  rst_expand/14(out6) -> reg14/2
  din_expand/14(out6) -> reg14/1
  en_expand/13(out7) -> reg13/3
  rst_expand/13(out7) -> reg13/2
  din_expand/13(out7) -> reg13/1
  en_expand/12(out8) -> reg12/3
  rst_expand/12(out8) -> reg12/2
  din_expand/12(out8) -> reg12/1
  en_expand/11(out9) -> reg11/3
  rst_expand/11(out9) -> reg11/2
  din_expand/11(out9) -> reg11/1
  en_expand/10(out10) -> reg10/3
  rst_expand/10(out10) -> reg10/2
  din_expand/10(out10) -> reg10/1
  en_expand/9(out11) -> reg9/3
  rst_expand/9(out11) -> reg9/2
  din_expand/9(out11) -> reg9/1
  en_expand/8(out12) -> reg8/3
  rst_expand/8(out12) -> reg8/2
  din_expand/8(out12) -> reg8/1
  en_expand/7(out13) -> reg7/3
  rst_expand/7(out13) -> reg7/2
  din_expand/7(out13) -> reg7/1
  en_expand/6(out14) -> reg6/3
  rst_expand/6(out14) -> reg6/2
  din_expand/6(out14) -> reg6/1
  en_expand/5(out15) -> reg5/3
  rst_expand/5(out15) -> reg5/2
  din_expand/5(out15) -> reg5/1
  en_expand/4(out16) -> reg4/3
  rst_expand/4(out16) -> reg4/2
  din_expand/4(out16) -> reg4/1
  en_expand/3(out17) -> reg3/3
  rst_expand/3(out17) -> reg3/2
  din_expand/3(out17) -> reg3/1
  en_expand/2(out18) -> reg2/3
  rst_expand/2(out18) -> reg2/2
  din_expand/2(out18) -> reg2/1
  en_expand/1(msb_out19) -> reg1/3
  rst_expand/1(msb_out19) -> reg1/2
  din_expand/1(msb_out19) -> reg1/1
  en/1 -> en_expand/1(bus_in)
  rst/1 -> rst_expand/1(bus_in)
  din/1 -> din_expand/1(bus_in)
